simulink model "am"  (R2023b)
settings: Solver=VariableStepAuto  StartTime=0.0  StopTime=1  MaxStep=0.00001  RelTol=1e-3
libraries: dspfdesign x1
settings Model: Creator=Хз_переименуюсь  LastModifiedBy=Хз_переименуюсь

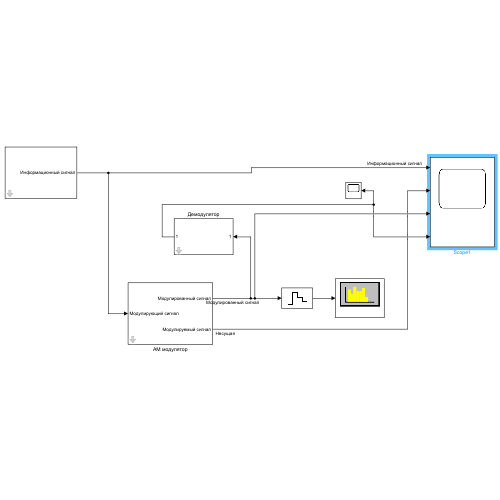
[thumbnail: Simulink's stored preview of the top-level diagram]
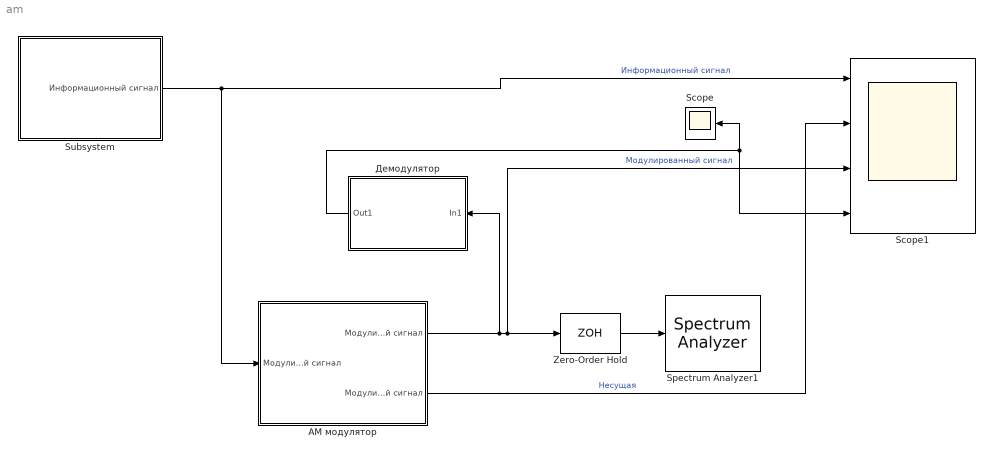
== system am ==
  AM модулятор : Subsystem  mask{Fc=300, mu=0.5}
      mask prompts: Fc "Частота несущей, Гц"; mu "Порядок модуляции mu"
  Scope : Scope
  Scope1 : Scope  NumInputPorts=4
  Spectrum Analyzer1 : SpectrumAnalyzer  WindowPosition=[1.000000,41.000000,1539.000000,940.000000,]  ScopeFrameLocation=window  FrequencySpan=Start and stop frequencies  Span=1000  StartFrequency=0  StopFrequency=500  YLimits=[-155.98829104,-14.50794531]
      settings: OpenAtSimulationStart=off
  Subsystem : Subsystem  mask{F1=20, F2=40, F3=60, F4=100}
      mask prompts: F1 "Частота1, Гц"; F2 "Частота1, Гц"; F3 "Частота3, Гц"; F4 "Частота4, Гц"
      mask DialogControl asdfsfdg Prompt: Parameters
  Zero-Order Hold : ZeroOrderHold  SampleTime=1e-3
  Демодулятор : Subsystem  mask{frq=300}
      mask prompts: frq "Частота несущей"
  wires:
  Subsystem/1(Информационный сигнал) -> AM модулятор/1(Модулирующий сигнал), Scope1/1  "Информационный сигнал"
  AM модулятор/1(Модулированный сигнал) -> Демодулятор/1(In1), Zero-Order Hold/1, Scope1/3  "Модулированный сигнал"
  Zero-Order Hold/1 -> Spectrum Analyzer1/1
  AM модулятор/2(Модулируемый сигнал) -> Scope1/2  "Несущая"
  Демодулятор/1(Out1) -> Scope1/4, Scope/1

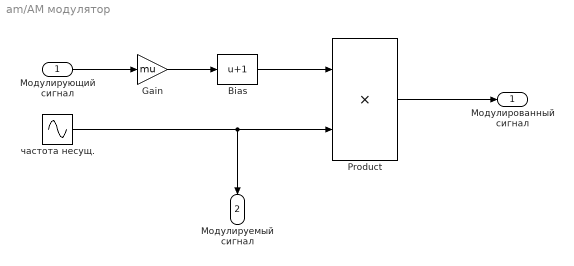
== system am/AM модулятор ==
  Модулирующий сигнал : Inport
  Bias : Bias  Bias=1  SaturateOnIntegerOverflow=off
  Gain : Gain  Gain=mu
  Product : Product
  частота несущ. : Sin  Frequency=2*pi*Fc  Phase=pi/2  SampleTime=0
  Модулированный сигнал : Outport
  Модулируемый сигнал : Outport  Port=2
  wires:
  Модулирующий сигнал/1 -> Gain/1
  Product/1 -> Модулированный сигнал/1
  Gain/1 -> Bias/1
  частота несущ./1 -> Product/2, Модулируемый сигнал/1
  Bias/1 -> Product/1

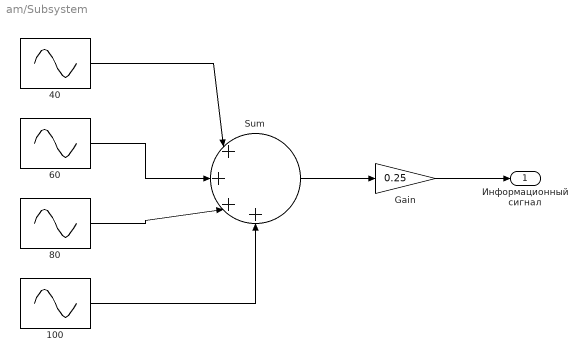
== system am/Subsystem ==
  100 : Sin  Frequency=2*pi*F4  SampleTime=0
  40 : Sin  Frequency=2*pi*F1  SampleTime=0
  60 : Sin  Frequency=2*pi*F2  SampleTime=0
  80 : Sin  Frequency=2*pi*F3  SampleTime=0
  Gain : Gain  Gain=0.25
  Sum : Sum  Inputs=|++++
  Информационный сигнал : Outport
  wires:
  40/1 -> Sum/1
  60/1 -> Sum/2
  80/1 -> Sum/3
  Sum/1 -> Gain/1
  100/1 -> Sum/4
  Gain/1 -> Информационный сигнал/1

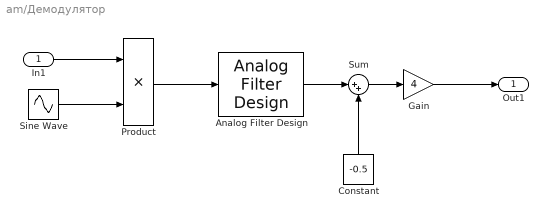
== system am/Демодулятор ==
  In1 : Inport
  Analog Filter Design : dspfdesign/Analog Filter Design  method=Butterworth  filttype=Lowpass  N=16  Wlo=2*pi*frq  Whi=80  Rp=2  Rs=40
  Constant : Constant  Value=-0.5
  Gain : Gain  Gain=4
  Product : Product
  Sine Wave : Sin  Frequency=2*pi*frq  Phase=pi/2  SampleTime=0
  Sum : Sum  Inputs=|++
  Out1 : Outport
  wires:
  Gain/1 -> Out1/1
  Sum/1 -> Gain/1
  Sine Wave/1 -> Product/2
  Product/1 -> Analog Filter Design/1
  Analog Filter Design/1 -> Sum/1
  Constant/1 -> Sum/2
  In1/1 -> Product/1
